simulink model "tire_brake_deceleration"  (R2024a)
settings: Solver=ode1  StartTime=0.0  StopTime=10  FixedStep=0.001  RelTol=1e-3
PostLoadFcn:
  | , if any(exist('dsrtsu_mdlpostloadfcn', 'file') == [2, 3, 6]), try dsrtsu_mdlpostloadfcn('Execute', bdroot); catch fprintf('Error in PostLoadFcn (dsrtsu_mdlpostloadfcn) for model "%s":\n %s\n', bdroot, lasterr); end, end,
InitFcn:
  | , if any(exist('rtifpga_mdlclblib', 'file') ~= 0), rtifpga_mdlclblib('Init', bdroot); end,
values from neighbouring files (symbols this model uses):
  a = 1.2    [init_parameters.m]
  Ap = [0, 1, 0, 0 ... (first row only)    [init_parameters.m]
  As = Ap    [init_parameters.m]
  b = 1.6    [init_parameters.m]
  Bp = [0 ... (first row only)    [init_parameters.m]
  Bs = [0, 0, 0 ... (first row only)    [init_parameters.m]
  c_max = 4000    [init_parameters.m]
  c_min = 500    [init_parameters.m]
  cf = 3.5e3    (= 3500)    [init_parameters.m]
  Cp = eye(4)    [init_parameters.m]
  cr = 3.5e3    (= 3500)    [init_parameters.m]
  Cs = Cp    [init_parameters.m]
  Dp = zeros(4, 1)    [init_parameters.m]
  Ds = zeros(4, 3)    [init_parameters.m]
  g = 9.81    [init_parameters.m]
  h = 0.5    [init_parameters.m]
  K = lqr(As, B_control, Q, R)    [init_parameters.m]
  kf = 35e3    (= 35000)    [init_parameters.m]
  kr = 35e3    (= 35000)    [init_parameters.m]
  m = 1600    [init_parameters.m]
  mu = 0.4    [init_parameters.m]
libraries: simulink x4
Description:
  | Standard RTI1401 template.
  | Supported MATLAB version:  R2024a.
settings Model: Tag=RTI1401  DSRTSU_INTERNAL_RTI_VER=640  DSRTSU_INTERNAL_RTI_TYPE=rti1401  RTICANMMDATA=struct('GeneralSetupData',struct('modelroot','C:\Users\VM-User\Desktop\MigrationScripts','generalsettings',struct('filesettings',struct('destfolder',struct('Name','RTICANMM_FILES','Check',1),'buildfolder',struct('Name','.','Check',1),'AbsDestfolder',struct('Name','C:\Users\VM-User\Desktop\MigrationScripts\RTICANMM_FILES'),'AbsBuildfolder',struct('Name','C:\Users\VM-User\Desktop\MigrationScripts'))),'options',struct('addpaths',1,'rmpaths',1,'addtrcexclusion',true,'cannavigator',struct('checkmonitoring',0),'show_usrtrc',0,'use_usrtrc',0),'advanced',struct('options',ones(1,100)),'MPSetup',{{}},'RTI',struct('Type','RTI1401','Ver','7.17','Date','02-Nov-2021'),'modelname','','block','untitled'))  DSRTSU_INTERNAL_RTIFPGA=210  DSRTSU_INTERNAL_RTISTBM_VER=24.1  Creator=ivanv  LastModifiedBy=ivanv
settings SolverCC: AlgebraicLoopSolver=TrustRegion
settings DataIOCC: ReturnWorkspaceOutputs=off
settings OptimizationCC: BlockReduction=off  OptimizeBlockIOStorage=off  BufferReuse=off  ReuseModelBlockBuffer=off  GlobalBufferReuse=off  ExpressionFolding=off  LocalBlockOutputs=off  OptimizeDataStoreBuffers=off  BusAssignmentInplaceUpdate=off
settings DebuggingCC: UnconnectedInputMsg=warning  UnconnectedOutputMsg=warning  UnconnectedLineMsg=warning  PregeneratedLibrarySubsystemCodeDiagnostic=none  ArithmeticOperatorsInVariantConditions=warning
settings HardwareCC: ProdBitPerPointer=32  ProdBitPerSizeT=32  ProdBitPerPtrDiffT=32  ProdLargestAtomicInteger=Integer  ProdEndianess=BigEndian  ProdWordSize=32  ProdLongLongMode=on  ProdHWDeviceType=Custom Processor->Custom  TargetIntDivRoundTo=Zero  TargetEndianess=BigEndian  TargetHWDeviceType=Custom Processor->Custom
settings ModelReferenceCC: EnableRefExpFcnMdlSchedulingChecks=on  EnableParallelModelReferenceBuilds=on  ParallelModelReferenceMATLABWorkerInit=Load Top Model
settings SFSimCC: SimUseLocalCustomCode=off  MATLABDynamicMemAlloc=off  CustomCodeUndefinedFunction=UseInterfaceOnly
settings RTWCC: Description=dSPACE DS1401 Hardware Platform  SystemTargetFile=rti1401.tlc  MakeCommand=make_rti  TemplateMakefile=rti1401.tmf  RTWUseLocalCustomCode=off  GPUComputeCapability=3.5  DLArmComputeVersion=19.05
settings CodeAppCC: StateflowObjectComments=on
settings STFCustomTargetCC: TargetLangStandard=C89/C90 (ANSI)  ParMdlRefBuildCompliant=on  MatFileLogging=on  GRTInterface=off  UseToolchainInfoCompliant=off  SystemTargetFile=rti1401.tlc
settings GRTTargetCC: TargetLangStandard=C89/C90 (ANSI)  CompOptLevelCompliant=off  ConcurrentExecutionCompliant=off  CombineOutputUpdateFcns=off  CPPClassGenCompliant=off  UseToolchainInfoCompliant=off
settings ConfigComp: CovMetricSettings=dswe

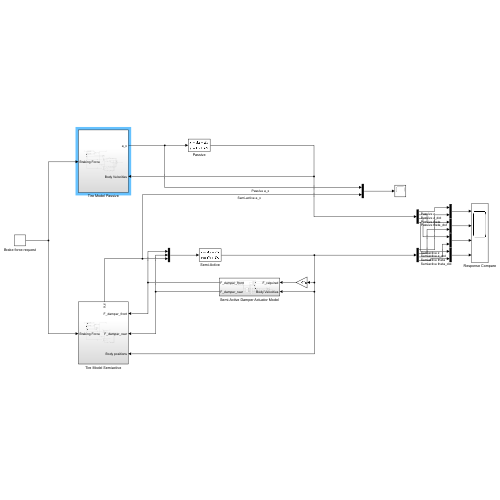
[thumbnail: Simulink's stored preview of the top-level diagram]
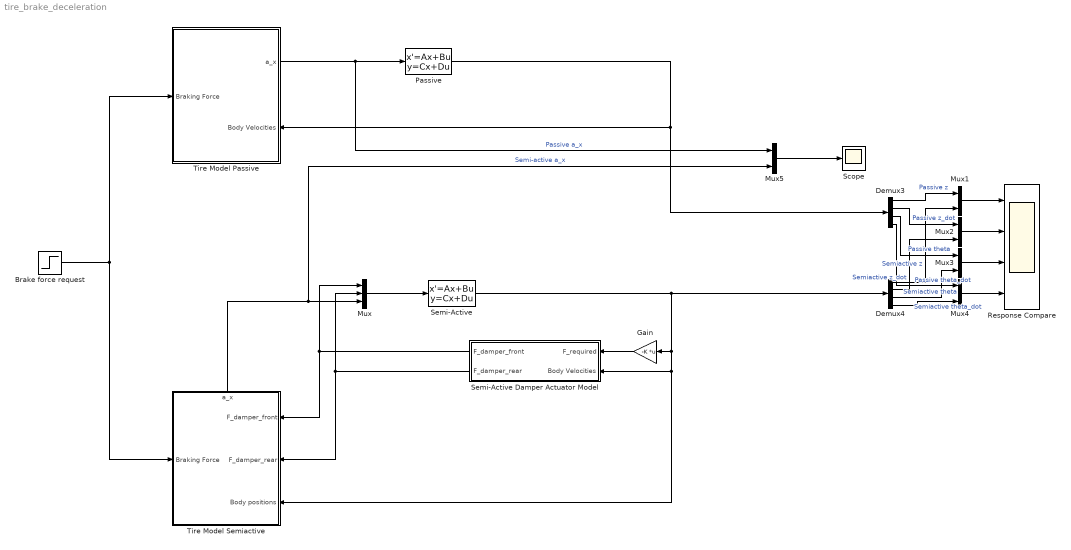
== system tire_brake_deceleration ==
  Brake force request : Step  After=5000  SampleTime=0
  Demux3 : Demux
  Demux4 : Demux
  Gain : Gain  Gain=-K  Multiplication=Matrix(K*u)
  Mux : Mux  Inputs=3
  Mux{1..5} (5 alike) : Mux  Inputs=2
  Passive : StateSpace  A=Ap  B=Bp  C=Cp  D=Dp  InitialCondition=0
  Response Compare : Scope  NumInputPorts=4
  Scope : Scope
  Semi-Active : StateSpace  A=As  B=Bs  C=Cs  D=Ds  InitialCondition=0
  Semi-Active Damper Actuator Model : Subsystem
  Tire Model Passive : Subsystem
      settings: PortSchema="{\"entries\":[{\"content\":{\"sides\":[{\"content\":{\"connectorIds\":[\"Out1\",\"In1\"]},\"type\":\"ConnectorPlacement.EquallySpacedRectSide\",\"uuid\":\"f5993897-d871-41ac-90d7-fcf2b0c913db\"},{\"content\":{\"connectorIds\":[\"In2\"],\"side\":\"RIGHT\"},\"type\":\"ConnectorPlacement.EquallySpacedRectSide\",\"uuid\":\"589172a9-dfdb-4c44-b449-b4a239416c46\"},{\"content\":{\"side\":\"TOP\"},\"type\":\"ConnectorPlacement.EquallySpacedRectSide\",\"uuid\":\"41693c0a-1ec9-4bdb-92e9-cee87a3d136d\"}]},\"type\":\"ConnectorPlacement.EquallySpacedConnector\",\"uuid\":\"38e33c93-264c-4c7b-b702-177705216bb6\"}],\"packageUris\":[\"http://schema.mathworks.com/mf0/Connector/R2020b\"],\"version\":\"1.0\"}"
  Tire Model Semiactive : Subsystem
      settings: PortSchema="{\"entries\":[{\"content\":{\"sides\":[{\"content\":{\"connectorIds\":[\"In1\",\"In2\",\"In3\"]},\"type\":\"ConnectorPlacement.EquallySpacedRectSide\",\"uuid\":\"f5993897-d871-41ac-90d7-fcf2b0c913db\"},{\"content\":{\"connectorIds\":[\"In4\"],\"side\":\"RIGHT\"},\"type\":\"ConnectorPlacement.EquallySpacedRectSide\",\"uuid\":\"589172a9-dfdb-4c44-b449-b4a239416c46\"},{\"content\":{\"connectorIds\":[\"Out1\"],\"side\":\"TOP\"},\"type\":\"ConnectorPlacement.EquallySpacedRectSide\",\"uuid\":\"41693c0a-1ec9-4bdb-92e9-cee87a3d136d\"}]},\"type\":\"ConnectorPlacement.EquallySpacedConnector\",\"uuid\":\"38e33c93-264c-4c7b-b702-177705216bb6\"}],\"packageUris\":[\"http://schema.mathworks.com/mf0/Connector/R2020b\"],\"version\":\"1.0\"}"
  wires:
  Passive/1 -> Demux3/1, Tire Model Passive/1(Body Velocities)
  Mux/1 -> Semi-Active/1
  Semi-Active/1 -> Demux4/1, Tire Model Semiactive/3(Body positions), Semi-Active Damper Actuator Model/2(Body Velocities), Gain/1
  Mux1/1 -> Response Compare/1
  Mux2/1 -> Response Compare/2
  Mux3/1 -> Response Compare/3
  Mux4/1 -> Response Compare/4
  Demux3/1 -> Mux1/1  "Passive z"
  Demux4/1 -> Mux1/2  "Semiactive z"
  Demux3/2 -> Mux2/1  "Passive z_dot"
  Demux4/2 -> Mux2/2  "Semiactive z_dot"
  Demux3/3 -> Mux3/1  "Passive theta"
  Demux4/3 -> Mux3/2  "Semiactive theta"
  Demux3/4 -> Mux4/1  "Passive theta_dot"
  Demux4/4 -> Mux4/2  "Semiactive theta_dot"
  Gain/1 -> Semi-Active Damper Actuator Model/1(F_required)
  Semi-Active Damper Actuator Model/1(F_damper_front) -> Tire Model Semiactive/1(F_damper_front), Mux/1
  Semi-Active Damper Actuator Model/2(F_damper_rear) -> Tire Model Semiactive/2(F_damper_rear), Mux/2
  Brake force request/1 -> Tire Model Semiactive/4(Braking Force), Tire Model Passive/2(Braking Force)
  Tire Model Semiactive/1(a_x) -> Mux5/2, Mux/3  "Semi-active a_x"
  Tire Model Passive/1(a_x) -> Mux5/1, Passive/1  "Passive a_x"
  Mux5/1 -> Scope/1

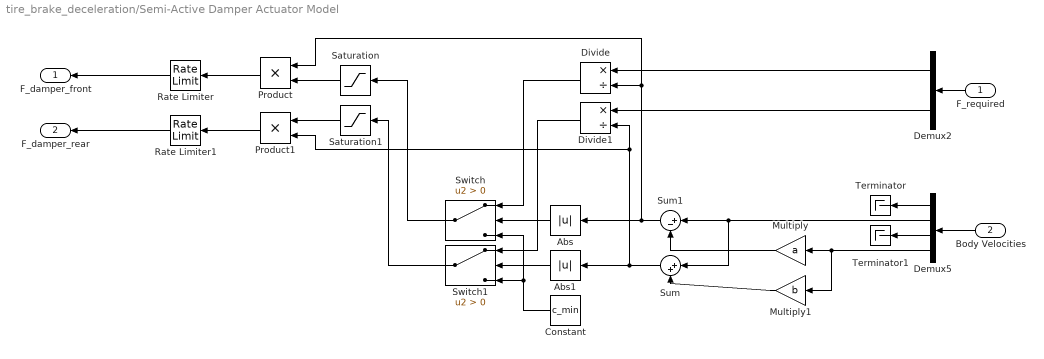
== system tire_brake_deceleration/Semi-Active Damper Actuator Model ==
  F_required : Inport
  Body Velocities : Inport  Port=2
  Abs : Abs  SaturateOnIntegerOverflow=off
  Abs1 : Abs  SaturateOnIntegerOverflow=off
  Constant : Constant  Value=c_min
  Demux2 : Demux  Outputs=2
  Demux5 : Demux
  Divide : Product  Inputs=*/
  Divide1 : Product  Inputs=*/
  Multiply : Gain  Gain=a
  Multiply1 : Gain  Gain=b
  Product : Product
  Product1 : Product
  Rate Limiter : RateLimiter  RisingSlewLimit=175000  FallingSlewLimit=-175000  SampleTimeMode=inherited
  Rate Limiter1 : RateLimiter  RisingSlewLimit=175000  FallingSlewLimit=-175000  SampleTimeMode=inherited
  Saturation : Saturate  UpperLimit=c_max  LowerLimit=c_min
  Saturation1 : Saturate  UpperLimit=c_max  LowerLimit=c_min
  Sum : Sum  Inputs=|++
  Sum1 : Sum  Inputs=|+-
  Switch : Switch  Criteria=u2 > Threshold  SaturateOnIntegerOverflow=off  InputSameDT=off
  Switch1 : Switch  Criteria=u2 > Threshold  SaturateOnIntegerOverflow=off  InputSameDT=off
  Terminator : Terminator
  Terminator1 : Terminator
  F_damper_front : Outport
  F_damper_rear : Outport  Port=2
  wires:
  Constant/1 -> Switch/3, Switch1/3
  Demux5/1 -> Terminator/1
  Demux5/4 -> Multiply1/1, Multiply/1
  Sum1/1 -> Abs/1, Product/1, Divide/2
  Demux2/1 -> Divide/1
  Body Velocities/1 -> Demux5/1
  Saturation/1 -> Product/2
  Demux5/2 -> Sum1/1, Sum/1
  Abs/1 -> Switch/2
  Product/1 -> Rate Limiter/1
  Switch1/1 -> Saturation1/1
  Divide/1 -> Switch/1
  Switch/1 -> Saturation/1
  Sum/1 -> Abs1/1, Product1/2, Divide1/2
  Demux2/2 -> Divide1/1
  Rate Limiter1/1 -> F_damper_rear/1
  Multiply1/1 -> Sum/2
  F_required/1 -> Demux2/1
  Abs1/1 -> Switch1/2
  Saturation1/1 -> Product1/1
  Multiply/1 -> Sum1/2
  Demux5/3 -> Terminator1/1
  Product1/1 -> Rate Limiter1/1
  Divide1/1 -> Switch1/1
  Rate Limiter/1 -> F_damper_front/1

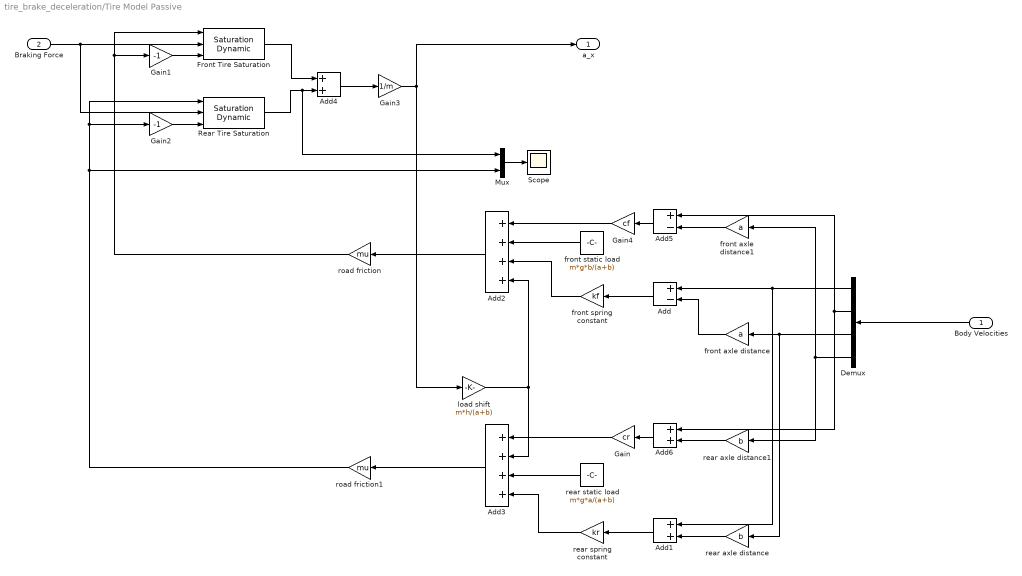
== system tire_brake_deceleration/Tire Model Passive ==
  Body Velocities : Inport
  Braking Force : Inport  Port=2
  Add : Sum  Inputs=+-
  Add1 : Sum
  Add2 : Sum  Inputs=++++
  Add3 : Sum  Inputs=++++
  Add4 : Sum
  Add5 : Sum  Inputs=+-
  Add6 : Sum
  Demux : Demux
  Front Tire Saturation : simulink/Discontinuities/Saturation Dynamic  OutMin=[]  OutMax=[]  OutDataTypeStr=Inherit: Same as second input  OutDataType=fixdt(1, 16)  OutScaling=2^-10  DoSatur=off
  Gain : Gain  Gain=cr
  Gain1 : Gain  Gain=-1
  Gain2 : Gain  Gain=-1
  Gain3 : Gain  Gain=1/m
  Gain4 : Gain  Gain=cf
  Mux : Mux  Inputs=2
  Rear Tire Saturation : simulink/Discontinuities/Saturation Dynamic  OutMin=[]  OutMax=[]  OutDataTypeStr=Inherit: Same as second input  OutDataType=fixdt(1, 16)  OutScaling=2^-10  DoSatur=off
  Scope : Scope
  front axle distance : Gain  Gain=a
  front axle distance1 : Gain  Gain=a
  front spring constant : Gain  Gain=kf
  front static load : Constant  Value=m*g*b/(a+b)
  load shift : Gain  Gain=m*h/(a+b)
  rear axle distance : Gain  Gain=b
  rear axle distance1 : Gain  Gain=b
  rear spring constant : Gain  Gain=kr
  rear static load : Constant  Value=m*g*a/(a+b)
  road friction : Gain  Gain=mu
  road friction1 : Gain  Gain=mu
  a_x : Outport
  wires:
  Demux/2 -> Add5/1, Add6/1
  Gain2/1 -> Rear Tire Saturation/3
  rear static load/1 -> Add3/3
  Gain3/1 -> load shift/1, a_x/1
  Front Tire Saturation/1 -> Add4/1
  Add/1 -> front spring constant/1
  rear axle distance/1 -> Add1/2
  Add2/1 -> road friction/1
  front static load/1 -> Add2/2
  rear spring constant/1 -> Add3/4
  load shift/1 -> Add2/4, Add3/2
  front axle distance/1 -> Add/2
  front spring constant/1 -> Add2/3
  road friction/1 -> Front Tire Saturation/1, Gain1/1
  Add4/1 -> Gain3/1
  Body Velocities/1 -> Demux/1
  Demux/1 -> Add1/1, Add/1
  Add6/1 -> Gain/1
  Gain1/1 -> Front Tire Saturation/3
  Add5/1 -> Gain4/1
  Add3/1 -> road friction1/1
  Add1/1 -> rear spring constant/1
  Braking Force/1 -> Front Tire Saturation/2, Rear Tire Saturation/2
  Demux/3 -> front axle distance/1, rear axle distance/1
  front axle distance1/1 -> Add5/2
  rear axle distance1/1 -> Add6/2
  Demux/4 -> front axle distance1/1, rear axle distance1/1
  Gain/1 -> Add3/1
  Gain4/1 -> Add2/1
  Mux/1 -> Scope/1
  Rear Tire Saturation/1 -> Mux/1, Add4/2
  road friction1/1 -> Mux/2, Rear Tire Saturation/1, Gain2/1

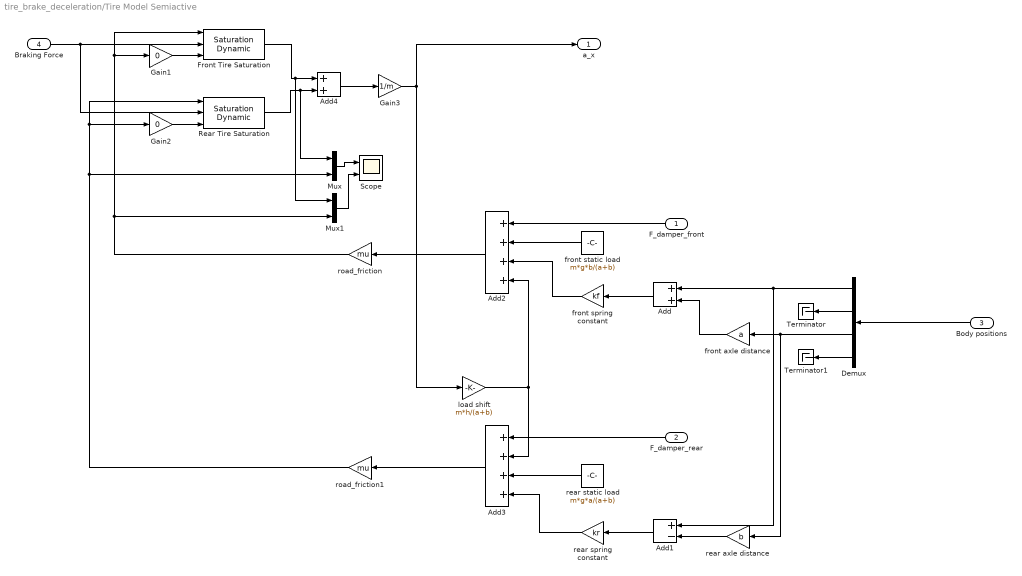
== system tire_brake_deceleration/Tire Model Semiactive ==
  F_damper_front : Inport
  F_damper_rear : Inport  Port=2
  Body positions : Inport  Port=3
  Braking Force : Inport  Port=4
  Add : Sum
  Add1 : Sum  Inputs=+-
  Add2 : Sum  Inputs=++++
  Add3 : Sum  Inputs=++++
  Add4 : Sum
  Demux : Demux
  Front Tire Saturation : simulink/Discontinuities/Saturation Dynamic  OutMin=[]  OutMax=[]  OutDataTypeStr=Inherit: Same as second input  OutDataType=fixdt(1, 16)  OutScaling=2^-10  DoSatur=off
  Gain1 : Gain  Gain=0
  Gain2 : Gain  Gain=0
  Gain3 : Gain  Gain=1/m
  Mux : Mux  Inputs=2
  Mux1 : Mux  Inputs=2
  Rear Tire Saturation : simulink/Discontinuities/Saturation Dynamic  OutMin=[]  OutMax=[]  OutDataTypeStr=Inherit: Same as second input  OutDataType=fixdt(1, 16)  OutScaling=2^-10  DoSatur=off
  Scope : Scope  NumInputPorts=2
  Terminator : Terminator
  Terminator1 : Terminator
  front axle distance : Gain  Gain=a
  front spring constant : Gain  Gain=kf
  front static load : Constant  Value=m*g*b/(a+b)
  load shift : Gain  Gain=m*h/(a+b)
  rear axle distance : Gain  Gain=b
  rear spring constant : Gain  Gain=kr
  rear static load : Constant  Value=m*g*a/(a+b)
  road_friction : Gain  Gain=mu
  road_friction1 : Gain  Gain=mu
  a_x : Outport
  wires:
  Demux/3 -> rear axle distance/1, front axle distance/1
  Braking Force/1 -> Rear Tire Saturation/2, Front Tire Saturation/2
  Add1/1 -> rear spring constant/1
  Add3/1 -> road_friction1/1
  F_damper_front/1 -> Add2/1
  Gain1/1 -> Front Tire Saturation/3
  F_damper_rear/1 -> Add3/1
  road_friction1/1 -> Gain2/1, Rear Tire Saturation/1, Mux/2
  Demux/1 -> Add/1, Add1/1
  Body positions/1 -> Demux/1
  Add4/1 -> Gain3/1
  road_friction/1 -> Gain1/1, Front Tire Saturation/1, Mux1/2
  front spring constant/1 -> Add2/3
  front axle distance/1 -> Add/2
  load shift/1 -> Add3/2, Add2/4
  rear spring constant/1 -> Add3/4
  front static load/1 -> Add2/2
  Add2/1 -> road_friction/1
  rear axle distance/1 -> Add1/2
  Add/1 -> front spring constant/1
  Demux/4 -> Terminator1/1
  Front Tire Saturation/1 -> Mux1/1, Add4/1
  Gain3/1 -> a_x/1, load shift/1
  rear static load/1 -> Add3/3
  Gain2/1 -> Rear Tire Saturation/3
  Demux/2 -> Terminator/1
  Rear Tire Saturation/1 -> Mux/1, Add4/2
  Mux/1 -> Scope/1
  Mux1/1 -> Scope/2
